simulink model "Autonomous_Test"  (R2023b)
settings: Solver=FixedStepDiscrete  StartTime=0.0  StopTime=20  FixedStep=0.020  MaxStep=0.020  RelTol=1e-3
undefined symbols (not defined in the file or in its folder): All_Paths_Ref_Poses_Blue, All_Paths_Ref_Poses_Red, Auto_Deploy_Intake_Time, Auto_Path_01, Auto_Path_02, Auto_Path_03, Auto_Path_04, Auto_Path_05, Auto_Path_06, Auto_Path_07, Auto_Path_Chooser, Auto_Shoot_Time, DiscIntNeverNeededParam, sim_IC_x, sim_IC_y, Spline_Capture_Radius, Spline_Lookahead_Dist, Spline_Velocity_Axis, t_sample, test_cases
libraries: simulink x6, simulink_extras x1
settings Model: PauseTimes=9.10  Creator=ander  LastModifiedBy=ander

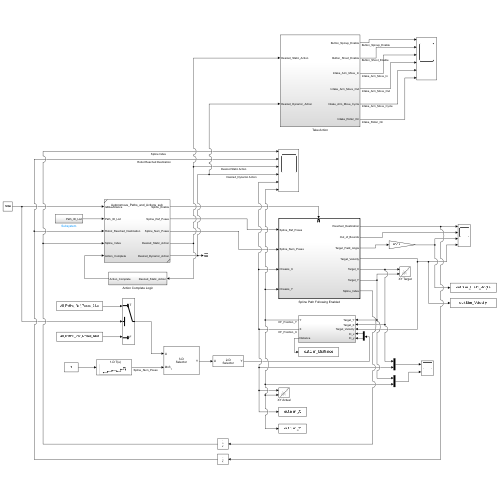
[thumbnail: Simulink's stored preview of the top-level diagram]
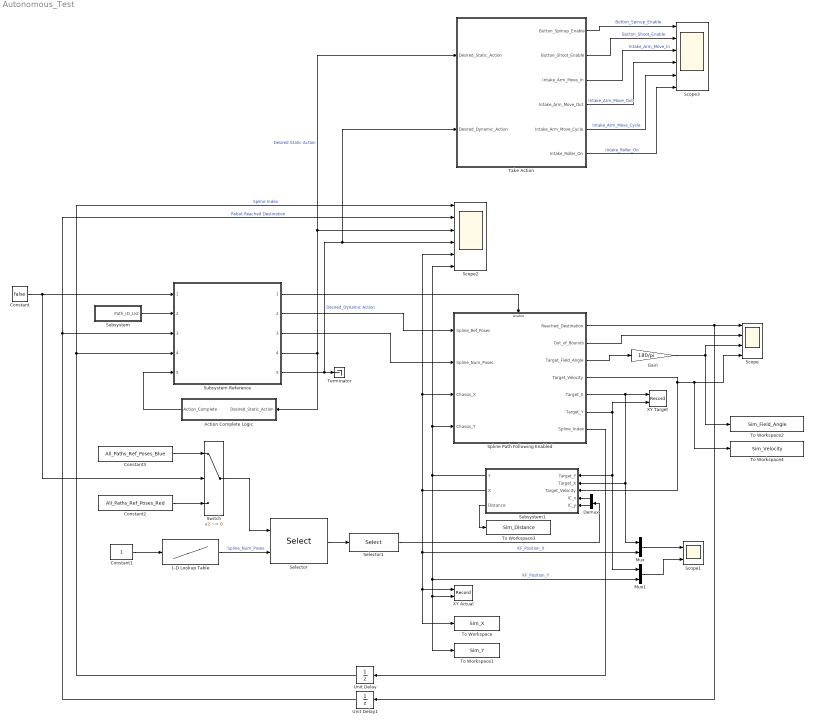
== system Autonomous_Test ==
  1-D Lookup Table : Lookup_n-D  NumberOfTableDimensions=1  BreakpointsSpecification=Even spacing  BreakpointsForDimension1=[-5:5]  Table=test_cases  InterpMethod=Flat  InternalRulePriority=Speed  RndMeth=Simplest
  Action Complete Logic : Subsystem
  Constant : Constant  Value=false
  Constant1 : Constant
  Constant2 : Constant  Value=All_Paths_Ref_Poses_Red
  Constant3 : Constant  Value=All_Paths_Ref_Poses_Blue
  Demux : Demux  Outputs=2
  Gain : Gain  Gain=180/pi
  Mux : Mux  Inputs=2
  Mux1 : Mux  Inputs=2
  Scope : Scope  NumInputPorts=4
  Scope1 : Scope  NumInputPorts=2
  Scope2 : Scope  NumInputPorts=6
  Scope3 : Scope  NumInputPorts=6
  Selector : Selector  NumberOfDimensions=3  InputPortWidth=3  IndexOptions=Select all,Select all,Index vector (port)  Indices=[1 3],1,1  OutputSizes=1,1,1
  Selector1 : Selector  NumberOfDimensions=2  InputPortWidth=3  IndexOptions=Index vector (dialog),Index vector (dialog)  Indices=[1],[1 2]  OutputSizes=1,1
  Spline Path Following Enabled : Subsystem
  Subsystem : Subsystem
  Subsystem Reference : Subsystem  ReferencedSubsystem=Autonomous_Paths_and_Actions_sub
  Subsystem1 : Subsystem
  Switch : Switch  Criteria=u2 ~= 0  SaturateOnIntegerOverflow=off  InputSameDT=off
  Take Action : Subsystem
  Terminator : Terminator
  To Workspace : ToWorkspace  VariableName=Sim_X  SaveFormat=Structure With Time  SampleTime=0.02
      settings: Save2DSignal=2-D array (concatenate along first dimension)
  To Workspace1 : ToWorkspace  VariableName=Sim_Y  SaveFormat=Structure With Time  SampleTime=0.02
      settings: Save2DSignal=2-D array (concatenate along first dimension)
  To Workspace2 : ToWorkspace  VariableName=Sim_Field_Angle  SaveFormat=Structure With Time  SampleTime=0.02
      settings: Save2DSignal=2-D array (concatenate along first dimension)
  To Workspace3 : ToWorkspace  VariableName=Sim_Distance  SaveFormat=Structure With Time  SampleTime=0.02
      settings: Save2DSignal=2-D array (concatenate along first dimension)
  To Workspace4 : ToWorkspace  VariableName=Sim_Velocity  SaveFormat=Structure With Time  SampleTime=0.02
      settings: Save2DSignal=2-D array (concatenate along first dimension)
  Unit Delay : UnitDelay  SampleTime=-1  HasFrameUpgradeWarning=on
  Unit Delay1 : UnitDelay  SampleTime=-1  HasFrameUpgradeWarning=on
  XY Actual : Record  FileSettingsInternal="{\"entries\":[{\"content\":{\"excelSettings\":{\"content\":{},\"type\":\"Streamout.ExcelSettings\"}},\"type\":\"Streamout.FileSettingStorage\",\"uuid\":\"\"}],\"packageUris\":[\"http:\\/\\/schema.mathworks.com\\/mf0\\/streamout_blocks\\/R2020a\"],\"version\":\"1.0\"}"  Layout=[1 1]  SignalsInternal="{\"entries\":[{\"content\":{\"signals\":[{\"content\":{\"blockPath\":[],\"dimensions\":[1,1],\"domain\":\"\",\"lineColor\":\"#0072bd\",\"plots\":[1],\"port\":1,\"sid\":[\"\"],\"signalID\":7153,\"signalName\":\"KF_Position_X\"},\"type\":\"RecordBlkView.Signal\",\"uuid\":\"\"},{\"content\":{\"blockPath\":[],\"dimensions\":[1,1],\"domain\":\"\",\"lineColor\":\"#d95319\",\"plots\":[1],\"port\":2,\"sid\":[\"\"],\"signalID\":7157,\"signalName\":\"KF_Position_Y\"},\"type\":\"RecordBlkView.Signal\",\"uuid\":\"\"}]},\"type\":\"RecordBlkView.InputSignals\",\"uuid\":\"\"}],\"packageUris\":[\"http:\\/\\/schema.mathworks.com\\/mf0\\/streamout_blocks\\/R2020a\"],\"version\":\"1.0\"}"  VisualizationBindings="{\"xyplotplugin\":{\"info\":[{\"series\":[{\"bindingParametersList\":[{\"parameter\":\"X-Axis\",\"signalID\":7153,\"signalName\":\"KF_Position_X\"},{\"parameter\":\"Y-Axis\",\"signalID\":7157,\"signalName\":\"KF_Position_Y\"}],\"seriesID\":60078}],\"subplotID\":1}]}}"  CompatibilityTag=XY
  XY Target : Record  FileSettingsInternal="{\"entries\":[{\"content\":{\"excelSettings\":{\"content\":{},\"type\":\"Streamout.ExcelSettings\"}},\"type\":\"Streamout.FileSettingStorage\",\"uuid\":\"\"}],\"packageUris\":[\"http:\\/\\/schema.mathworks.com\\/mf0\\/streamout_blocks\\/R2020a\"],\"version\":\"1.0\"}"  Layout=[1 1]  SignalsInternal="{\"entries\":[{\"content\":{\"signals\":[{\"content\":{\"blockPath\":[],\"dimensions\":[1,1],\"domain\":\"\",\"lineColor\":\"#edb120\",\"plots\":[1],\"port\":1,\"sid\":[\"\"],\"signalID\":7161,\"signalName\":\"Spline Path Following Enabled:5\"},\"type\":\"RecordBlkView.Signal\",\"uuid\":\"\"},{\"content\":{\"blockPath\":[],\"dimensions\":[1,1],\"domain\":\"\",\"lineColor\":\"#7e2f8e\",\"plots\":[1],\"port\":2,\"sid\":[\"\"],\"signalID\":7165,\"signalName\":\"Spline Path Following Enabled:6\"},\"type\":\"RecordBlkView.Signal\",\"uuid\":\"\"}]},\"type\":\"RecordBlkView.InputSignals\",\"uuid\":\"\"}],\"packageUris\":[\"http:\\/\\/schema.mathworks.com\\/mf0\\/streamout_blocks\\/R2020a\"],\"version\":\"1.0\"}"  VisualizationBindings="{\"xyplotplugin\":{\"info\":[{\"series\":[{\"bindingParametersList\":[{\"parameter\":\"X-Axis\",\"signalID\":7161,\"signalName\":\"Spline Path Following Enabled:5\"},{\"parameter\":\"Y-Axis\",\"signalID\":7165,\"signalName\":\"Spline Path Following Enabled:6\"}],\"seriesID\":18176}],\"subplotID\":1}]}}"  CompatibilityTag=XY
  wires:
  Spline Path Following Enabled/5(Target_X) -> Mux/1, Subsystem1/2(Target_X), XY Target/1
  Spline Path Following Enabled/6(Target_Y) -> Mux1/1, Subsystem1/1(Target_Y), XY Target/2
  Subsystem1/2(X) -> Scope2/5, Spline Path Following Enabled/3(Chassis_X), Mux/2, XY Actual/1, To Workspace/1  "KF_Position_X"
  Spline Path Following Enabled/1(Reached_Destination) -> Scope/1, Unit Delay1/1
  Subsystem1/1(Y) -> Mux1/2, To Workspace1/1, XY Actual/2, Scope2/6, Spline Path Following Enabled/4(Chassis_Y)  "KF_Position_Y"
  Spline Path Following Enabled/4(Target_Velocity) -> Subsystem1/3(Target_Velocity), To Workspace4/1, Scope/4
  Spline Path Following Enabled/3(Target_Field_Angle) -> Gain/1
  Gain/1 -> To Workspace2/1, Scope/3
  Spline Path Following Enabled/2(Out_of_Bounds) -> Scope/2
  Mux1/1 -> Scope1/2
  Subsystem1/3(Distance) -> To Workspace3/1
  Mux/1 -> Scope1/1
  Subsystem Reference/2 -> Spline Path Following Enabled/1(Spline_Ref_Poses)
  Subsystem Reference/3 -> Spline Path Following Enabled/2(Spline_Num_Poses)
  Spline Path Following Enabled/7(Spline_Index) -> Unit Delay/1
  Unit Delay/1 -> Subsystem Reference/4, Scope2/1  "Spline Index"
  Unit Delay1/1 -> Subsystem Reference/3, Scope2/2  "Robot Reached Destination"
  Selector/1 -> Selector1/1
  Demux/1 -> Subsystem1/4(IC_x)
  Demux/2 -> Subsystem1/5(IC_y)
  Selector1/1 -> Demux/1
  Subsystem Reference/4 -> Action Complete Logic/1(Desired_Static_Action), Take Action/1(Desired_Static_Action), Scope2/3  "Desired Static Action"
  1-D Lookup Table/1 -> Selector/2  "Spline_Num_Poses"
  Constant1/1 -> 1-D Lookup Table/1
  Subsystem Reference/1 -> Spline Path Following Enabled/Enable
  Subsystem Reference/5 -> Take Action/2(Desired_Dynamic_Action), Scope2/4, Terminator/1  "Desired_Dynamic Action"
  Action Complete Logic/1(Action_Complete) -> Subsystem Reference/5
  Subsystem/1(Path_ID_List) -> Subsystem Reference/2
  Constant/1 -> Switch/2, Subsystem Reference/1
  Switch/1 -> Selector/1
  Constant2/1 -> Switch/3
  Constant3/1 -> Switch/1
  Take Action/1(Button_Spinup_Enable) -> Scope3/1  "Button_Spinup_Enable"
  Take Action/2(Button_Shoot_Enable) -> Scope3/2  "Button_Shoot_Enable"
  Take Action/3(Intake_Arm_Move_In) -> Scope3/3  "Intake_Arm_Move_In"
  Take Action/4(Intake_Arm_Move_Out) -> Scope3/4  "Intake_Arm_Move_Out"
  Take Action/5(Intake_Arm_Move_Cycle) -> Scope3/5  "Intake_Arm_Move_Cycle"
  Take Action/6(Intake_Roller_On) -> Scope3/6  "Intake_Roller_On"

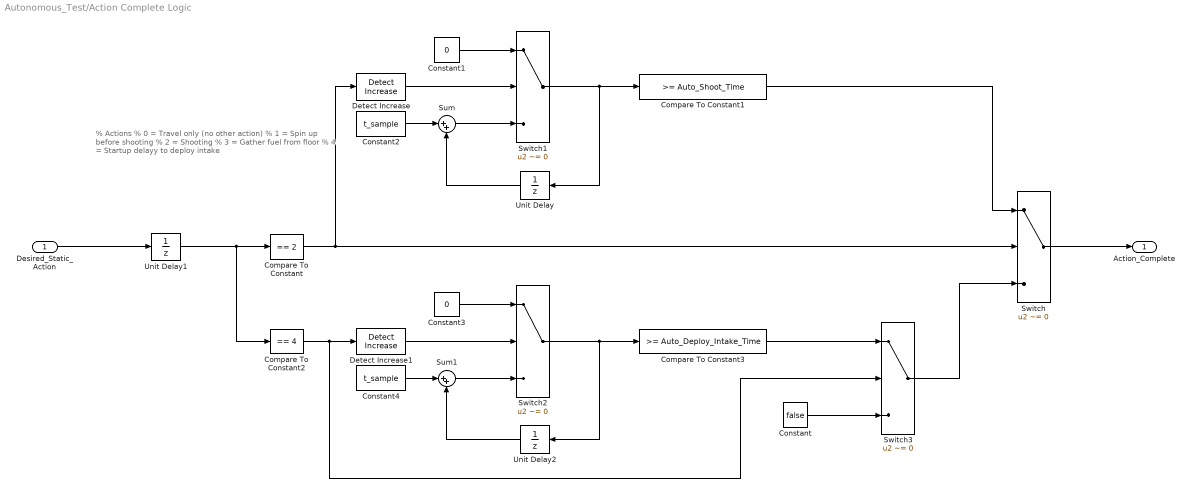
== system Autonomous_Test/Action Complete Logic ==
  note: % Actions
      | % 0 = Travel only (no other action)
      | % 1 = Spin up before shooting
      | % 2 = Shooting
      | % 3 = Gather fuel from floor
      | % 4 = Startup delayy to deploy intake
  Desired_Static_Action : Inport
  Compare To Constant : simulink/Logic and Bit Operations/Compare To Constant  relop===  const=2  OutDataTypeStr=boolean
  Compare To Constant1 : simulink/Logic and Bit Operations/Compare To Constant  relop=>=  const=Auto_Shoot_Time  OutDataTypeStr=boolean
  Compare To Constant2 : simulink/Logic and Bit Operations/Compare To Constant  relop===  const=4  OutDataTypeStr=boolean
  Compare To Constant3 : simulink/Logic and Bit Operations/Compare To Constant  relop=>=  const=Auto_Deploy_Intake_Time  OutDataTypeStr=boolean
  Constant : Constant  Value=false
  Constant1 : Constant  Value=0
  Constant2 : Constant  Value=t_sample
  Constant3 : Constant  Value=0
  Constant4 : Constant  Value=t_sample
  Detect Increase : simulink/Logic and Bit Operations/Detect Increase  vinit=0.0  OutDataTypeStr=boolean
  Detect Increase1 : simulink/Logic and Bit Operations/Detect Increase  vinit=0.0  OutDataTypeStr=boolean
  Sum : Sum  Inputs=|++
  Sum1 : Sum  Inputs=|++
  Switch{,1..3} (4 alike) : Switch  Criteria=u2 ~= 0  SaturateOnIntegerOverflow=off  InputSameDT=off
  Unit Delay : UnitDelay  SampleTime=-1  HasFrameUpgradeWarning=on
  Unit Delay1 : UnitDelay  SampleTime=-1  HasFrameUpgradeWarning=on
  Unit Delay2 : UnitDelay  SampleTime=-1  HasFrameUpgradeWarning=on
  Action_Complete : Outport
  wires:
  Desired_Static_Action/1 -> Unit Delay1/1
  Compare To Constant/1 -> Detect Increase/1, Switch/2
  Switch/1 -> Action_Complete/1
  Detect Increase/1 -> Switch1/2
  Constant1/1 -> Switch1/1
  Sum/1 -> Switch1/3
  Constant2/1 -> Sum/1
  Switch1/1 -> Compare To Constant1/1, Unit Delay/1
  Unit Delay/1 -> Sum/2
  Compare To Constant1/1 -> Switch/1
  Unit Delay1/1 -> Compare To Constant2/1, Compare To Constant/1
  Constant4/1 -> Sum1/1
  Unit Delay2/1 -> Sum1/2
  Sum1/1 -> Switch2/3
  Detect Increase1/1 -> Switch2/2
  Switch2/1 -> Compare To Constant3/1, Unit Delay2/1
  Constant3/1 -> Switch2/1
  Compare To Constant2/1 -> Switch3/2, Detect Increase1/1
  Switch3/1 -> Switch/3
  Compare To Constant3/1 -> Switch3/1
  Constant/1 -> Switch3/3

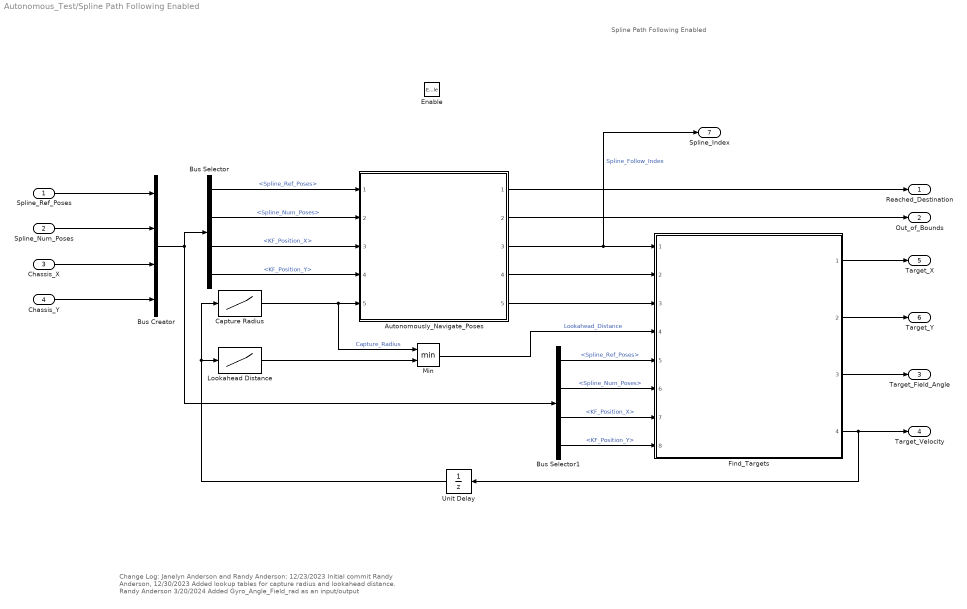
== system Autonomous_Test/Spline Path Following Enabled ==
  note: Spline Path Following Enabled
  note: Change Log:
      | Janelyn Anderson and Randy Anderson: 12/23/2023
      | Initial commit
      | Randy Anderson, 12/30/2023
      | Added lookup tables for capture radius and lookahead distance.
      | Randy Anderson 3/20/2024
      | Added Gyro_Angle_Field_rad as an input/output
  Spline_Ref_Poses : Inport
  Spline_Num_Poses : Inport  Port=2
  Chassis_X : Inport  Port=3
  Chassis_Y : Inport  Port=4
  Enable : EnablePort  StatesWhenEnabling=reset  PropagateVarSize=During execution
  Autonomously_Navigate_Poses : Subsystem  ReferencedSubsystem=Autonomously_Navigate_Poses
  Bus Creator : BusCreator  Inputs=4
  Bus Selector : BusSelector  OutputSignals=Spline_Ref_Poses,Spline_Num_Poses,KF_Position_X,KF_Position_Y
  Bus Selector1 : BusSelector  OutputSignals=Spline_Ref_Poses,Spline_Num_Poses,KF_Position_X,KF_Position_Y
  Capture Radius : Lookup_n-D  NumberOfTableDimensions=1  BreakpointsForDimension1=Spline_Velocity_Axis  Table=Spline_Capture_Radius  ExtrapMethod=Clip  InternalRulePriority=Speed  RndMeth=Simplest
  Find_Targets : Subsystem  ReferencedSubsystem=Find_Target_Position_Velocity_Heading
  Lookahead Distance : Lookup_n-D  NumberOfTableDimensions=1  BreakpointsForDimension1=Spline_Velocity_Axis  Table=Spline_Lookahead_Dist  ExtrapMethod=Clip  InternalRulePriority=Speed  RndMeth=Simplest
  Min : MinMax  Inputs=2
  Unit Delay : UnitDelay  SampleTime=-1  HasFrameUpgradeWarning=on
  Reached_Destination : Outport
  Out_of_Bounds : Outport  Port=2
  Target_Field_Angle : Outport  Port=3
  Target_Velocity : Outport  Port=4
  Target_X : Outport  Port=5
  Target_Y : Outport  Port=6
  Spline_Index : Outport  Port=7
  wires:
  Autonomously_Navigate_Poses/5 -> Find_Targets/3
  Autonomously_Navigate_Poses/4 -> Find_Targets/2
  Autonomously_Navigate_Poses/3 -> Spline_Index/1, Find_Targets/1  "Spline_Follow_Index"
  Find_Targets/4 -> Target_Velocity/1, Unit Delay/1
  Spline_Ref_Poses/1 -> Bus Creator/1
  Spline_Num_Poses/1 -> Bus Creator/2
  Chassis_X/1 -> Bus Creator/3
  Chassis_Y/1 -> Bus Creator/4
  Bus Creator/1 -> Bus Selector1/1, Bus Selector/1
  Bus Selector/2 -> Autonomously_Navigate_Poses/2  "<Spline_Num_Poses>"
  Bus Selector/1 -> Autonomously_Navigate_Poses/1  "<Spline_Ref_Poses>"
  Bus Selector1/2 -> Find_Targets/6  "<Spline_Num_Poses>"
  Bus Selector1/1 -> Find_Targets/5  "<Spline_Ref_Poses>"
  Bus Selector/3 -> Autonomously_Navigate_Poses/3  "<KF_Position_X>"
  Bus Selector/4 -> Autonomously_Navigate_Poses/4  "<KF_Position_Y>"
  Bus Selector1/3 -> Find_Targets/7  "<KF_Position_X>"
  Bus Selector1/4 -> Find_Targets/8  "<KF_Position_Y>"
  Capture Radius/1 -> Autonomously_Navigate_Poses/5, Min/1  "Capture_Radius"
  Unit Delay/1 -> Lookahead Distance/1, Capture Radius/1
  Lookahead Distance/1 -> Min/2
  Min/1 -> Find_Targets/4  "Lookahead_Distance"
  Find_Targets/1 -> Target_X/1
  Find_Targets/2 -> Target_Y/1
  Find_Targets/3 -> Target_Field_Angle/1
  Autonomously_Navigate_Poses/1 -> Reached_Destination/1
  Autonomously_Navigate_Poses/2 -> Out_of_Bounds/1

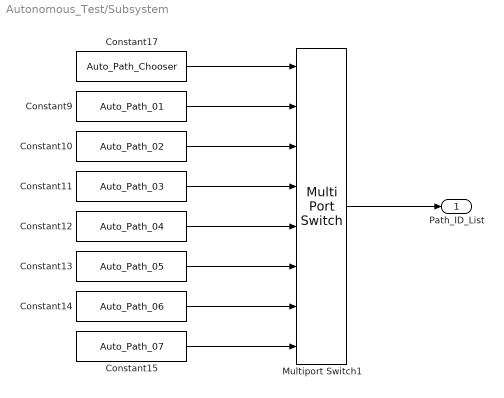
== system Autonomous_Test/Subsystem ==
  Constant10 : Constant  Value=Auto_Path_02
  Constant11 : Constant  Value=Auto_Path_03
  Constant12 : Constant  Value=Auto_Path_04
  Constant13 : Constant  Value=Auto_Path_05
  Constant14 : Constant  Value=Auto_Path_06
  Constant15 : Constant  Value=Auto_Path_07
  Constant17 : Constant  Value=Auto_Path_Chooser
  Constant9 : Constant  Value=Auto_Path_01
  Multiport Switch1 : MultiPortSwitch  Inputs=7  SaturateOnIntegerOverflow=off  InputSameDT=off
  Path_ID_List : Outport
  wires:
  Constant10/1 -> Multiport Switch1/3
  Constant14/1 -> Multiport Switch1/7
  Constant12/1 -> Multiport Switch1/5
  Constant13/1 -> Multiport Switch1/6
  Constant11/1 -> Multiport Switch1/4
  Constant15/1 -> Multiport Switch1/8
  Constant17/1 -> Multiport Switch1/1
  Constant9/1 -> Multiport Switch1/2
  Multiport Switch1/1 -> Path_ID_List/1

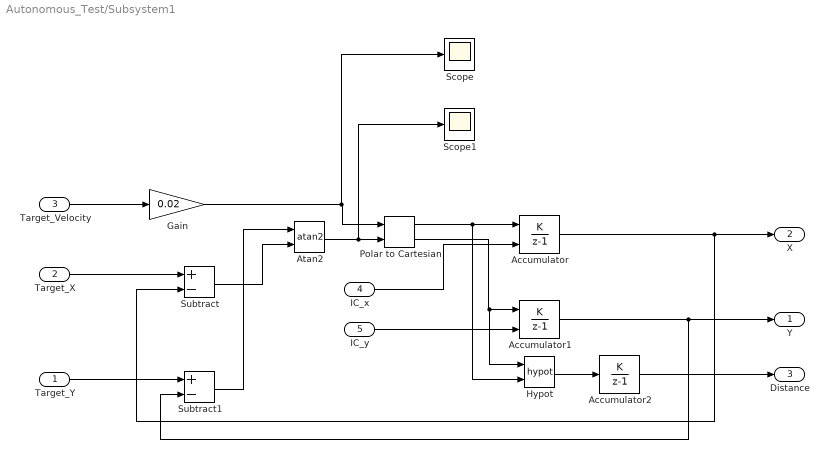
== system Autonomous_Test/Subsystem1 ==
  Target_Y : Inport
  Target_X : Inport  Port=2
  Target_Velocity : Inport  Port=3
  IC_x : Inport  Port=4
  IC_y : Inport  Port=5
  Accumulator : DiscreteIntegrator  IntegratorMethod=Accumulation: Forward Euler  InitialConditionSource=external  InitialCondition=sim_IC_x  SampleTime=-1  ICPrevOutput=DiscIntNeverNeededParam  ICPrevScaledInput=DiscIntNeverNeededParam
  Accumulator1 : DiscreteIntegrator  IntegratorMethod=Accumulation: Forward Euler  InitialConditionSource=external  InitialCondition=sim_IC_y  SampleTime=-1  ICPrevOutput=DiscIntNeverNeededParam  ICPrevScaledInput=DiscIntNeverNeededParam
  Accumulator2 : DiscreteIntegrator  IntegratorMethod=Accumulation: Forward Euler  SampleTime=-1  ICPrevOutput=DiscIntNeverNeededParam  ICPrevScaledInput=DiscIntNeverNeededParam
  Atan2 : Trigonometry  Operator=atan2
  Gain : Gain  Gain=0.02
  Hypot : Math  Operator=hypot
  Polar to Cartesian : simulink_extras/Transformations/Polar to Cartesian
  Scope : Scope
  Scope1 : Scope
  Subtract : Sum  Inputs=+-
  Subtract1 : Sum  Inputs=+-
  Y : Outport
  X : Outport  Port=2
  Distance : Outport  Port=3
  wires:
  Target_X/1 -> Subtract/1
  Target_Y/1 -> Subtract1/1
  Subtract1/1 -> Atan2/1
  Subtract/1 -> Atan2/2
  Atan2/1 -> Scope1/1, Polar to Cartesian/2
  Target_Velocity/1 -> Gain/1
  Polar to Cartesian/1 -> Hypot/2, Accumulator/1
  Gain/1 -> Scope/1, Polar to Cartesian/1
  Polar to Cartesian/2 -> Hypot/1, Accumulator1/1
  Accumulator1/1 -> Y/1, Subtract1/2
  Accumulator/1 -> X/1, Subtract/2
  Hypot/1 -> Accumulator2/1
  Accumulator2/1 -> Distance/1
  IC_x/1 -> Accumulator/2
  IC_y/1 -> Accumulator1/2

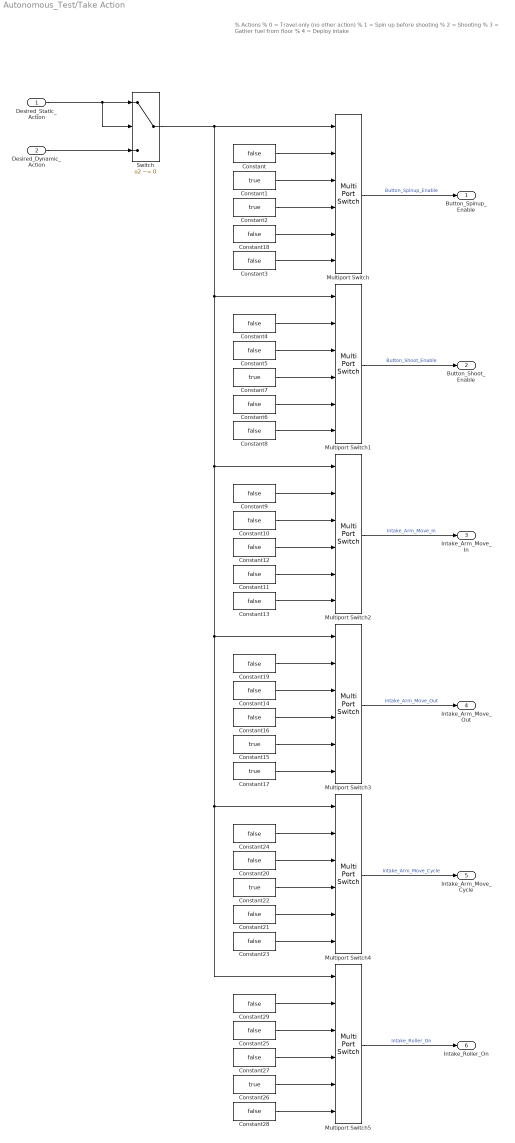
== system Autonomous_Test/Take Action ==
  note: % Actions
      | % 0 = Travel only (no other action)
      | % 1 = Spin up before shooting
      | % 2 = Shooting
      | % 3 = Gather fuel from floor
      | % 4 = Deploy intake
  Desired_Static_Action : Inport
  Desired_Dynamic_Action : Inport  Port=2
  Constant{,3..6,8..14,16,18..21,23..25,27..29} (23 alike) : Constant  Value=false
  Constant{1..2,7,15,17,22,26} (7 alike) : Constant  Value=true
  Multiport Switch{,1..5} (6 alike) : MultiPortSwitch  DataPortOrder=Zero-based contiguous  Inputs=5  zeroidx=on  SaturateOnIntegerOverflow=off  InputSameDT=off
  Switch : Switch  Criteria=u2 ~= 0  SaturateOnIntegerOverflow=off  InputSameDT=off
  Button_Spinup_Enable : Outport
  Button_Shoot_Enable : Outport  Port=2
  Intake_Arm_Move_In : Outport  Port=3
  Intake_Arm_Move_Out : Outport  Port=4
  Intake_Arm_Move_Cycle : Outport  Port=5
  Intake_Roller_On : Outport  Port=6
  wires:
  Multiport Switch/1 -> Button_Spinup_Enable/1  "Button_Spinup_Enable"
  Desired_Static_Action/1 -> Switch/2, Switch/1
  Desired_Dynamic_Action/1 -> Switch/3
  Switch/1 -> Multiport Switch1/1, Multiport Switch5/1, Multiport Switch4/1, Multiport Switch3/1, Multiport Switch2/1, Multiport Switch/1
  Constant/1 -> Multiport Switch/2
  Constant1/1 -> Multiport Switch/3
  Constant2/1 -> Multiport Switch/4
  Constant18/1 -> Multiport Switch/5
  Constant3/1 -> Multiport Switch/6
  Constant8/1 -> Multiport Switch1/6
  Constant6/1 -> Multiport Switch1/5
  Constant7/1 -> Multiport Switch1/4
  Constant5/1 -> Multiport Switch1/3
  Constant4/1 -> Multiport Switch1/2
  Constant11/1 -> Multiport Switch2/5
  Constant12/1 -> Multiport Switch2/4
  Constant9/1 -> Multiport Switch2/2
  Constant13/1 -> Multiport Switch2/6
  Constant10/1 -> Multiport Switch2/3
  Constant14/1 -> Multiport Switch3/3
  Constant17/1 -> Multiport Switch3/6
  Constant19/1 -> Multiport Switch3/2
  Constant16/1 -> Multiport Switch3/4
  Constant15/1 -> Multiport Switch3/5
  Constant21/1 -> Multiport Switch4/5
  Constant22/1 -> Multiport Switch4/4
  Constant24/1 -> Multiport Switch4/2
  Constant23/1 -> Multiport Switch4/6
  Constant20/1 -> Multiport Switch4/3
  Constant25/1 -> Multiport Switch5/3
  Constant28/1 -> Multiport Switch5/6
  Constant29/1 -> Multiport Switch5/2
  Constant27/1 -> Multiport Switch5/4
  Constant26/1 -> Multiport Switch5/5
  Multiport Switch1/1 -> Button_Shoot_Enable/1  "Button_Shoot_Enable"
  Multiport Switch2/1 -> Intake_Arm_Move_In/1  "Intake_Arm_Move_In"
  Multiport Switch3/1 -> Intake_Arm_Move_Out/1  "Intake_Arm_Move_Out"
  Multiport Switch4/1 -> Intake_Arm_Move_Cycle/1  "Intake_Arm_Move_Cycle"
  Multiport Switch5/1 -> Intake_Roller_On/1  "Intake_Roller_On"
